simulink model "LKA_Vision_TestBench"  (R2026a)
settings: Solver=ode4  StopTime=SCN.StopTime  FixedStep=0.005
undefined symbols (not defined in the file): LKA, ROAD, SCN, vehicle
libraries: sim3dautolib x1, sim3dcameralib x1, sim3dlib x1
Description:
  | Camera-in-the-loop LKA bench: Baja single-track plant, Unreal official LKA track, Simulation 3D Camera, switchable lane detector (YOLOP / team CNN / classic), wheel-speed and gyro models, LKA_Controller, ground-truth metrics.
settings Model: Creator=rithv  LastModifiedBy=rithv
settings DebuggingCC: AlgebraicLoopMsg=error

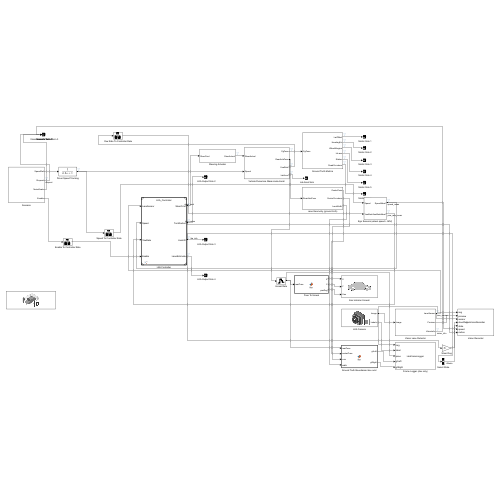
[thumbnail: Simulink's stored preview of the top-level diagram]
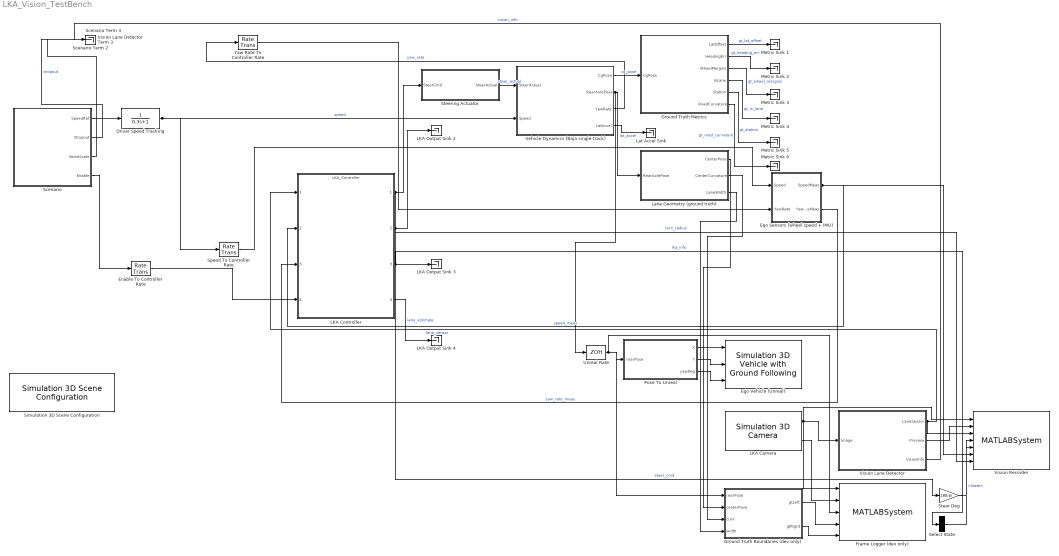
== system LKA_Vision_TestBench ==
  Driver Speed Tracking : TransferFcn  Numerator=1  Denominator=[0.3 1]
  Ego Sensors (wheel speed + IMU) : Subsystem
  Ego Vehicle (Unreal) : sim3dautolib/Simulation 3D Vehicle with Ground Following  Priority=-1  PassVehMesh=Muscle car  MeshPath=/MathWorksAutomotiveContent/Vehicles/Muscle/Meshes/SK_MuscleCar.SK_MuscleCar  TrackWidth=1.9  WheelBase=3  WheelRadius=0.35  VehColor=Red  CoordinateSystem=ISO8855  InitialPos=[0, 0, 0]  InitialRot=[0, 0, 0]  ActorName=LkaEgo  SampleTime=LKA.Ts  ActorType=SimulinkVehicle  ID=C  aMode=3  ActorTag=LkaEgo  CoordinateScheme=0  VehLightsControl=off  HeadlightColor=[ 1, 1, 1 ]  HighBeamIntensity=100000  LowBeamIntensity=60000  HighBeamConeAngle=70  LowBeamConeAngle=70  LeftHeadlightOrientation=[ 0, 0 ]  RightHeadlightOrientation=[ 0, 0 ]  BrakelightIntensity=500  ReverselightIntensity=500  SignallightIntensity=500  SignallightPeriod=1  SignalPulseWidth=50  TransformOutportEnabled=off
      settings: LibrarySourceBlock=drivingsim3d/Simulation 3D Vehicle with Ground Following
  Enable To Controller Rate : RateTransition  OutPortSampleTime=LKA.Ts
  Frame Logger (dev only) : MATLABSystem  System=LkaFrameLogger  Vision=LKA.Vision  Ts=LKA.Ts
      mask Type: LkaFrameLogger
  Ground Truth Boundaries (dev only) : MATLAB Function  TreatAsAtomicUnit=on
  Ground Truth Metrics : Subsystem
  LKA Camera : sim3dcameralib/Simulation 3D Camera  Priority=1  sensorTag=Sim3dSensor  sensorId=1  sensorName=Sim3dSensor  vehTagList={'Custom ...';'LkaEgo';'Scene Origin'}  vehTag=LkaEgo  CoordinateSystem=ISO8855  mountLoc=Origin  offsetFlag=on  tmountOffset=[LKA.Vision.Camera.X, LKA.Vision.Camera.Y, LKA.Vision.Camera.Height + LKA.Vision.Bench.MountZOffset]  extTmount=off  rmountOffset=[0, LKA.Vision.Bench.PitchSign * LKA.Vision.Camera.PitchDeg, 0]  extRmount=off  FocalLength=LKA.Vision.Camera.FocalLength  OpticalCenter=LKA.Vision.Camera.PrincipalPoint  ImageSize=LKA.Vision.Camera.ImageSize  RadialDistortion=[0, 0]  TangentialDistortion=[0, 0]  SensorSkew=0  VisualizeFieldOfView=off  FieldOfViewRange=61  DepthOutportEnabled=off  SemanticOutportEnabled=on  TransformOutportEnabled=off  SampleTime=LKA.Ts  mountPoint=[1.6 0 1.2]  mountOrientation=[0 8 0]  aMode=3  ID=1
      settings: LibrarySourceBlock=drivingsim3d/Simulation 3D Camera
  LKA Controller : ModelReference  ModelNameDialog=LKA_Controller  SimulationMode=Normal  ModelReferenceVersion=1.1
  LKA Output Sink 2 : Terminator
  LKA Output Sink 3 : Terminator
  LKA Output Sink 4 : Terminator
  Lane Geometry (ground truth) : Subsystem
  Lat Accel Sink : Terminator
  Metric Sink {1..6} (6 alike) : Terminator
  Pose To Unreal : MATLAB Function  TreatAsAtomicUnit=on
  Scenario : Subsystem
  Scenario Term 2 : Terminator
  Scenario Term 3 : Terminator
  Select State : BusSelector  OutputSignals=State
  Simulation 3D Scene Configuration : sim3dlib/Simulation 3D Scene Configuration  Priority=0  ProjectFormat=RoadRunner  SceneDesc=Straight road  ProjectName=D:\toolbox\shared\sim3d_projects\automotive_project_windows\UE\WindowsNoEditor\VehicleSimulation.exe  ScenePath=/Game/Maps/HwStrght  RoadRunnerProjectPath=E:\Abaja Labs\2026\LKA - Matlab\data\scenes\LKA\LKA.usd  EnableOpenDRIVE=off  vehTagList={'Custom';'Scene Origin'}  vehTag=Scene Origin  AttachedCameraRelativeTranslation=[0 0 0]  FreeCameraDefaultInitialTranslation=[-6, 0, 2]  AttachedCameraRelativeRotation=[0, -15, 0]  FreeCameraDefaultInitialRotation=[0, -15, 0]  ViewpointName=Custom  FreeCameraInitialTranslation=[0, 0, 0]  FreeCameraInitialRotation=[0, 0, 0]  OpVisEn=off  Ts=LKA.Ts  EnableWindow=on  EnableRemoteAccess=off  SimulationMode=CoSimulation  SimulateUsing=Interpreted execution  EnableAnimationRecording=off  OverrideDefaultRecording=off  AnimationRecordingFileName=sim3dAnimation.mat  AnimationRecordingInterval=[0 inf]  EnableWeather=off  SunAzimuth=90  SunAltitude=40.0  EnableGeospatialSun=off  Latitude=0  Longitude=0  Date=2023-01-01  Time=10:30:00  GeoTimeZone=-5.0  SunDaylightSaving=off  wind=1  clouds=10  EnableVolumetricClouds=off  CloudCoverage=0  CloudAltitude=6  fog=0  rain=0  RaindropsEffect=off  SnowDensity=0  EnableGeospatial=off  TilesetSource=Earth terrain  UseTrueOrigin=off  OriginHeight=200  OriginLatitude=40.744652  OriginLongitude=-73.988864  MapStyle=Aerial  AdditionalAssetIDs=[]  UseAdvancedSunSky=off  SolarTime=11  TimeZone=-5  Day=21  Month=9  Year=2022  UseDaylightSavingTime=on  DSTStartDay=10  DSTStartMonth=3  DSTEndDay=3  DSTEndMonth=11  DSTSwitchHour=2  sensorTag=MainCamera1  sensorId=1  sensorName=MainCamera1  mountLoc=Origin  offsetFlag=off  tmountOffset=[0, 0, 0]  rmountOffset=[0, 0, 0]  HorizontalResolution=1280  VerticalResolution=720  HorizontalFOV=60  mountPoint=[0 0 0]  mountOrientation=[0 0 0]  aMode=3  ID=1  GeoTrigger=Inactive  ViewNameList={'Custom'}  ViewTranslationList={'[0 0 0]'}  ViewRotationList={'[0 0 0]'}
      settings: LibrarySourceBlock=drivingsim3d/Simulation 3D Scene Configuration
  Speed To Controller Rate : RateTransition  OutPortSampleTime=LKA.Ts
  Steer Deg : Gain  Gain=180/pi
  Steering Actuator : Subsystem
  Unreal Rate : ZeroOrderHold  SampleTime=LKA.Ts
  Vehicle Dynamics (Baja single-track) : Subsystem
  Vision Lane Detector : Subsystem
  Vision Lane Detector Term 3 : Terminator
  Vision Recorder : MATLABSystem  System=LkaVisionRecorder  Vision=LKA.Vision  Ts=LKA.Ts
      mask Type: LkaVisionRecorder
  Yaw Rate To Controller Rate : RateTransition  OutPortSampleTime=LKA.Ts
  wires:
  Vehicle Dynamics (Baja single-track)/1(CgPose) -> Ground Truth Metrics/1(CgPose)  "cg_pose"
  Scenario/1(SpeedRef) -> Driver Speed Tracking/1
  Driver Speed Tracking/1 -> Vehicle Dynamics (Baja single-track)/2(Speed), Speed To Controller Rate/1  "speed"
  Scenario/4(Enable) -> Enable To Controller Rate/1
  Enable To Controller Rate/1 -> LKA Controller/4
  LKA Controller/1 -> Steering Actuator/1(SteerCmd), Steer Deg/1  "steer_cmd"
  LKA Controller/2 -> LKA Output Sink 2/1, Vision Recorder/7  "turn_radius"
  Vehicle Dynamics (Baja single-track)/2(RearAxlePose) -> Lane Geometry (ground truth)/1(RearAxlePose), Unreal Rate/1
  LKA Controller/3 -> LKA Output Sink 3/1, Select State/1  "lka_info"
  LKA Controller/4 -> LKA Output Sink 4/1  "lane_estimate"
  Steering Actuator/1(SteerActual) -> Vehicle Dynamics (Baja single-track)/1(SteerActual)  "steer_actual"
  Vehicle Dynamics (Baja single-track)/3(YawRate) -> Yaw Rate To Controller Rate/1  "yaw_rate"
  Vehicle Dynamics (Baja single-track)/4(LatAccel) -> Lat Accel Sink/1  "lat_accel"
  Ground Truth Metrics/1(LatOffset) -> Metric Sink 1/1  "gt_lat_offset"
  Ground Truth Metrics/2(HeadingErr) -> Metric Sink 2/1  "gt_heading_err"
  Ground Truth Metrics/3(WheelMargins) -> Metric Sink 3/1  "gt_wheel_margins"
  Ground Truth Metrics/4(InLane) -> Metric Sink 4/1  "gt_in_lane"
  Ground Truth Metrics/5(Station) -> Metric Sink 5/1  "gt_station"
  Ground Truth Metrics/6(RoadCurvature) -> Metric Sink 6/1  "gt_road_curvature"
  Scenario/2(Dropout) -> Scenario Term 2/1  "dropout"
  Scenario/3(NoiseScale) -> Scenario Term 3/1
  Unreal Rate/1 -> Pose To Unreal/1(rearPose), Ground Truth Boundaries (dev only)/1(rearPose), Frame Logger (dev only)/3
  Pose To Unreal/1(X) -> Ego Vehicle (Unreal)/1
  Pose To Unreal/2(Y) -> Ego Vehicle (Unreal)/2
  Pose To Unreal/3(yawDeg) -> Ego Vehicle (Unreal)/3
  LKA Camera/1 -> Vision Lane Detector/1(Image), Frame Logger (dev only)/1, Vision Recorder/1
  Vision Lane Detector/1(LaneSensor) -> LKA Controller/1, Vision Recorder/3  "lane_sensor"
  Lane Geometry (ground truth)/1(CenterPose) -> Ground Truth Boundaries (dev only)/2(centerPose)
  Lane Geometry (ground truth)/2(CenterCurvature) -> Ground Truth Boundaries (dev only)/3(curv)
  Lane Geometry (ground truth)/3(LaneWidth) -> Ground Truth Boundaries (dev only)/4(width)
  LKA Camera/2 -> Frame Logger (dev only)/2
  Ground Truth Boundaries (dev only)/1(gtLeft) -> Frame Logger (dev only)/4
  Ground Truth Boundaries (dev only)/2(gtRight) -> Frame Logger (dev only)/5
  Speed To Controller Rate/1 -> Ego Sensors (wheel speed + IMU)/1(Speed)
  Yaw Rate To Controller Rate/1 -> Ego Sensors (wheel speed + IMU)/2(YawRate)
  Ego Sensors (wheel speed + IMU)/1(SpeedMeas) -> LKA Controller/2, Vision Recorder/6  "speed_meas"
  Ego Sensors (wheel speed + IMU)/2(YawRateMeas) -> LKA Controller/3  "yaw_rate_meas"
  Vision Lane Detector/2(Preview) -> Vision Recorder/2
  Steer Deg/1 -> Vision Recorder/4
  Select State/1 -> Vision Recorder/5  "<State>"
  Vision Lane Detector/3(VisionInfo) -> Vision Lane Detector Term 3/1  "vision_info"

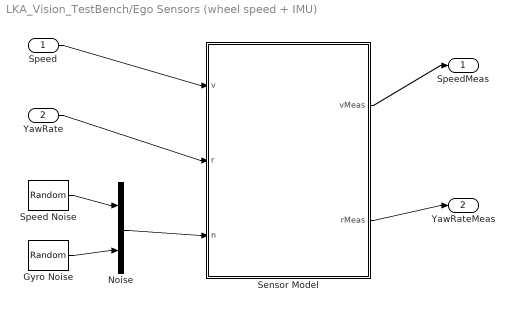
== system LKA_Vision_TestBench/Ego Sensors (wheel speed + IMU) ==
  Speed : Inport
  YawRate : Inport  Port=2
  Gyro Noise : RandomNumber  Seed=LKA.EgoSen.Seed(2)  SampleTime=LKA.Ts
  Noise : Mux  Inputs=2
  Sensor Model : MATLAB Function  TreatAsAtomicUnit=on
  Speed Noise : RandomNumber  Seed=LKA.EgoSen.Seed(1)  SampleTime=LKA.Ts
  SpeedMeas : Outport
  YawRateMeas : Outport  Port=2
  wires:
  Speed/1 -> Sensor Model/1(v)
  YawRate/1 -> Sensor Model/2(r)
  Speed Noise/1 -> Noise/1
  Gyro Noise/1 -> Noise/2
  Noise/1 -> Sensor Model/3(n)
  Sensor Model/1(vMeas) -> SpeedMeas/1
  Sensor Model/2(rMeas) -> YawRateMeas/1

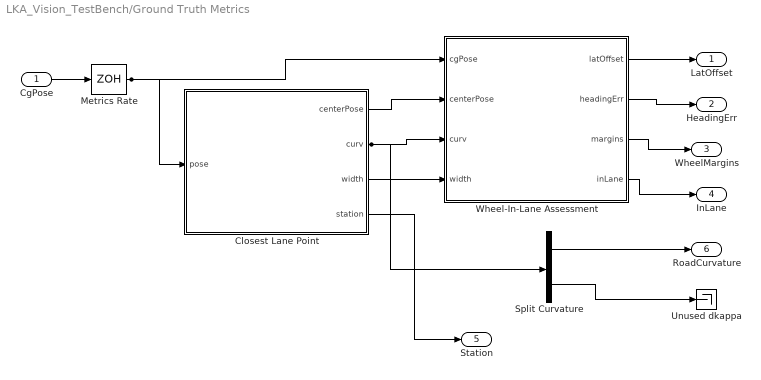
== system LKA_Vision_TestBench/Ground Truth Metrics ==
  CgPose : Inport
  Closest Lane Point : MATLAB Function  TreatAsAtomicUnit=on
  Metrics Rate : ZeroOrderHold  SampleTime=0.01
  Split Curvature : Demux  Outputs=2
  Unused dkappa : Terminator
  Wheel-In-Lane Assessment : MATLAB Function  TreatAsAtomicUnit=on
  LatOffset : Outport
  HeadingErr : Outport  Port=2
  WheelMargins : Outport  Port=3
  InLane : Outport  Port=4
  Station : Outport  Port=5
  RoadCurvature : Outport  Port=6
  wires:
  Wheel-In-Lane Assessment/2(headingErr) -> HeadingErr/1
  CgPose/1 -> Metrics Rate/1
  Metrics Rate/1 -> Wheel-In-Lane Assessment/1(cgPose), Closest Lane Point/1(pose)
  Closest Lane Point/1(centerPose) -> Wheel-In-Lane Assessment/2(centerPose)
  Closest Lane Point/4(station) -> Station/1
  Closest Lane Point/2(curv) -> Wheel-In-Lane Assessment/3(curv), Split Curvature/1
  Wheel-In-Lane Assessment/1(latOffset) -> LatOffset/1
  Closest Lane Point/3(width) -> Wheel-In-Lane Assessment/4(width)
  Wheel-In-Lane Assessment/3(margins) -> WheelMargins/1
  Wheel-In-Lane Assessment/4(inLane) -> InLane/1
  Split Curvature/1 -> RoadCurvature/1
  Split Curvature/2 -> Unused dkappa/1

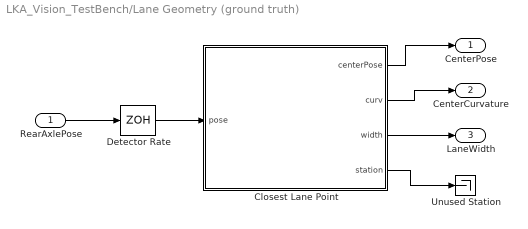
== system LKA_Vision_TestBench/Lane Geometry (ground truth) ==
  RearAxlePose : Inport
  Closest Lane Point : MATLAB Function  TreatAsAtomicUnit=on
  Detector Rate : ZeroOrderHold  SampleTime=LKA.Sen.Ts
  Unused Station : Terminator
  CenterPose : Outport
  CenterCurvature : Outport  Port=2
  LaneWidth : Outport  Port=3
  wires:
  RearAxlePose/1 -> Detector Rate/1
  Closest Lane Point/1(centerPose) -> CenterPose/1
  Detector Rate/1 -> Closest Lane Point/1(pose)
  Closest Lane Point/2(curv) -> CenterCurvature/1
  Closest Lane Point/3(width) -> LaneWidth/1
  Closest Lane Point/4(station) -> Unused Station/1

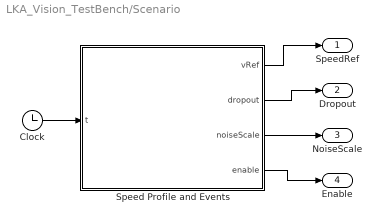
== system LKA_Vision_TestBench/Scenario ==
  Clock : Clock
  Speed Profile and Events : MATLAB Function  TreatAsAtomicUnit=on
  SpeedRef : Outport
  Dropout : Outport  Port=2
  NoiseScale : Outport  Port=3
  Enable : Outport  Port=4
  wires:
  Clock/1 -> Speed Profile and Events/1(t)
  Speed Profile and Events/1(vRef) -> SpeedRef/1
  Speed Profile and Events/2(dropout) -> Dropout/1
  Speed Profile and Events/3(noiseScale) -> NoiseScale/1
  Speed Profile and Events/4(enable) -> Enable/1

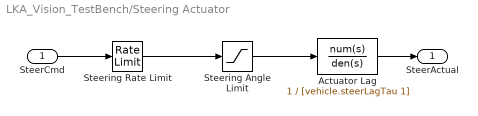
== system LKA_Vision_TestBench/Steering Actuator ==
  SteerCmd : Inport
  Actuator Lag : TransferFcn  Numerator=1  Denominator=[vehicle.steerLagTau 1]
  Steering Angle Limit : Saturate  UpperLimit=vehicle.maxSteerAngle  LowerLimit=-vehicle.maxSteerAngle
  Steering Rate Limit : RateLimiter  RisingSlewLimit=vehicle.maxSteerRate  FallingSlewLimit=-vehicle.maxSteerRate  SampleTimeMode=inherited
  SteerActual : Outport
  wires:
  SteerCmd/1 -> Steering Rate Limit/1
  Steering Rate Limit/1 -> Steering Angle Limit/1
  Steering Angle Limit/1 -> Actuator Lag/1
  Actuator Lag/1 -> SteerActual/1

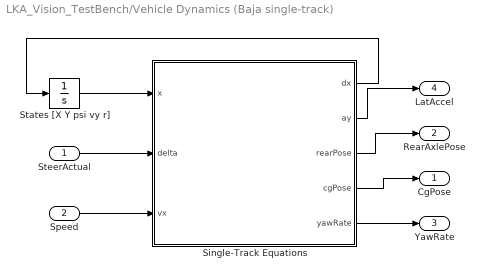
== system LKA_Vision_TestBench/Vehicle Dynamics (Baja single-track) ==
  SteerActual : Inport
  Speed : Inport  Port=2
  Single-Track Equations : MATLAB Function  TreatAsAtomicUnit=on
  States [X Y psi vy r] : Integrator  InitialCondition=SCN.X0
  CgPose : Outport
  RearAxlePose : Outport  Port=2
  YawRate : Outport  Port=3
  LatAccel : Outport  Port=4
  wires:
  States [X Y psi vy r]/1 -> Single-Track Equations/1(x)
  Single-Track Equations/5(yawRate) -> YawRate/1
  Single-Track Equations/1(dx) -> States [X Y psi vy r]/1
  SteerActual/1 -> Single-Track Equations/2(delta)
  Speed/1 -> Single-Track Equations/3(vx)
  Single-Track Equations/2(ay) -> LatAccel/1
  Single-Track Equations/3(rearPose) -> RearAxlePose/1
  Single-Track Equations/4(cgPose) -> CgPose/1

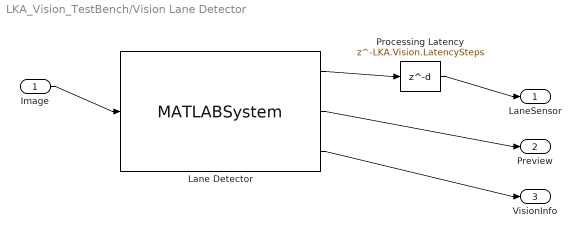
== system LKA_Vision_TestBench/Vision Lane Detector ==
  Image : Inport
  Lane Detector : MATLABSystem  System=LkaVisionLaneDetector  Vision=LKA.Vision  Ts=LKA.Ts
      mask Type: LkaVisionLaneDetector
  Processing Latency : Delay  DelayLength=LKA.Vision.LatencySteps  InitialCondition=0  SampleTime=LKA.Ts
  LaneSensor : Outport  OutDataTypeStr=Bus: LaneSensorBus
  Preview : Outport  Port=2
  VisionInfo : Outport  Port=3
  wires:
  Image/1 -> Lane Detector/1
  Lane Detector/1 -> Processing Latency/1
  Processing Latency/1 -> LaneSensor/1
  Lane Detector/2 -> Preview/1
  Lane Detector/3 -> VisionInfo/1

== matlab function LKA_Vision_TestBench/Vehicle Dynamics (Baja single-track)/Single-Track Equations ==
  data: x input; dx output; delta input; vx input; ay output; rearPose output; cgPose output; yawRate output; vehicle parameter
function [dx, ay, rearPose, cgPose, yawRate] = fcn(x, delta, vx, vehicle)
% Nonlinear bicycle model with saturating tyres (see lka_single_track_dynamics.m)
[dx, ay, rearPose] = lka_single_track_dynamics(x, delta, vx, vehicle);
cgPose = [x(1) x(2) x(3)];
yawRate = x(5);

== matlab function LKA_Vision_TestBench/Scenario/Speed Profile and Events ==
  data: t input; vRef output; dropout output; noiseScale output; enable output; SCN parameter
function [vRef, dropout, noiseScale, enable] = fcn(t, SCN)
% Driver speed profile v = min(V0 + a*t, VSet) and forced detector outages
vRef = min(SCN.V0 + SCN.Accel*t, SCN.VSet);
dropout = [0; 0];
for k = 1:size(SCN.Dropouts, 1)
    if t >= SCN.Dropouts(k,1) && t < SCN.Dropouts(k,2)
        side = SCN.Dropouts(k,3);
        if side == 1 || side == 3, dropout(1) = 1; end
        if side == 2 || side == 3, dropout(2) = 1; end
    end
end
noiseScale = SCN.NoiseScale;
enable = true;

== matlab function LKA_Vision_TestBench/Lane Geometry (ground truth)/Closest Lane Point ==
  data: pose input; centerPose output; curv output; width output; station output; ROAD parameter
function [centerPose, curv, width, station] = fcn(pose, ROAD)
% Foot point of the pose on the true lane centreline (windowed search, see lka_road_closest_point.m)
persistent idx
if isempty(idx), idx = 0; end
[centerPose, curv, width, station, idx] = lka_road_closest_point(pose(1), pose(2), idx, ...
    ROAD.s, ROAD.x, ROAD.y, ROAD.psi, ROAD.kappa, ROAD.dkappa, ROAD.width);

== matlab function LKA_Vision_TestBench/Pose To Unreal ==
  data: rearPose input; X output; Y output; yawDeg output; LKA parameter
function [X, Y, yawDeg] = fcn(rearPose, LKA)
% Track pose (OpenDRIVE / RoadRunner frame) -> Simulation 3D world inputs
[X, Y, yawDeg] = lka_pose_to_sim3d(rearPose, LKA.Vision.Bench.FrameMap);

== matlab function LKA_Vision_TestBench/Ground Truth Boundaries (dev only) ==
  data: rearPose input; gtLeft output; centerPose input; curv input; width input; gtRight output
function [gtLeft, gtRight] = fcn(rearPose, centerPose, curv, width)
% True ego-lane boundaries at the rear axle (benchmark ground truth)
[gtLeft, gtRight] = lka_lane_geometry(rearPose, centerPose, curv(1), curv(2), width);

== matlab function LKA_Vision_TestBench/Ground Truth Metrics/Closest Lane Point ==
  data: pose input; centerPose output; curv output; width output; station output; ROAD parameter
function [centerPose, curv, width, station] = fcn(pose, ROAD)
% Foot point of the pose on the true lane centreline (windowed search, see lka_road_closest_point.m)
persistent idx
if isempty(idx), idx = 0; end
[centerPose, curv, width, station, idx] = lka_road_closest_point(pose(1), pose(2), idx, ...
    ROAD.s, ROAD.x, ROAD.y, ROAD.psi, ROAD.kappa, ROAD.dkappa, ROAD.width);

== matlab function LKA_Vision_TestBench/Ground Truth Metrics/Wheel-In-Lane Assessment ==
  data: cgPose input; latOffset output; centerPose input; curv input; width input; headingErr output; margins output; inLane output; ROAD parameter; vehicle parameter
function [latOffset, headingErr, margins, inLane] = fcn(cgPose, centerPose, curv, width, ROAD, vehicle)
% True CG offset, heading error and tyre-edge-to-line margins (rulebook K.2.4)
[latOffset, headingErr, margins, inLane] = lka_ground_truth_metrics(cgPose, centerPose, curv, width, ROAD.lineWidth, vehicle);

== matlab function LKA_Vision_TestBench/Ego Sensors (wheel speed + IMU)/Sensor Model ==
  data: v input; vMeas output; r input; n input; rMeas output; LKA parameter
function [vMeas, rMeas] = fcn(v, r, n, LKA)
% Wheel-speed sensor and gyro with scale error, bias and noise (lka_ego_sensor_model.m)
[vMeas, rMeas] = lka_ego_sensor_model(v, r, n, LKA.EgoSen);
